simulink model "Emergency_Power_System"  (R2021b)
settings: Solver=FixedStepDiscrete  StartTime=0.0  StopTime=0.05  RelTol=1e-3
undefined symbols (not defined in the file): Ion, Lithium
libraries: spsSeriesRLCBranchLib x4, spsBatteryLib x1, spsBuckConverterLib x1, spsCurrentMeasurementLib x1, spsGroundLib x1, spsPWMGeneratorDCDCLib x1, spsVoltageMeasurementLib x1, spspowerguiLib x1
settings Model: Creator=KennyBoum-biha  LastModifiedBy=KennyBoum-biha

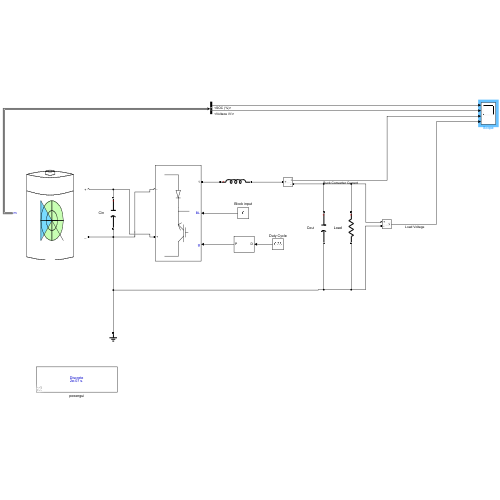
[thumbnail: Simulink's stored preview of the top-level diagram]
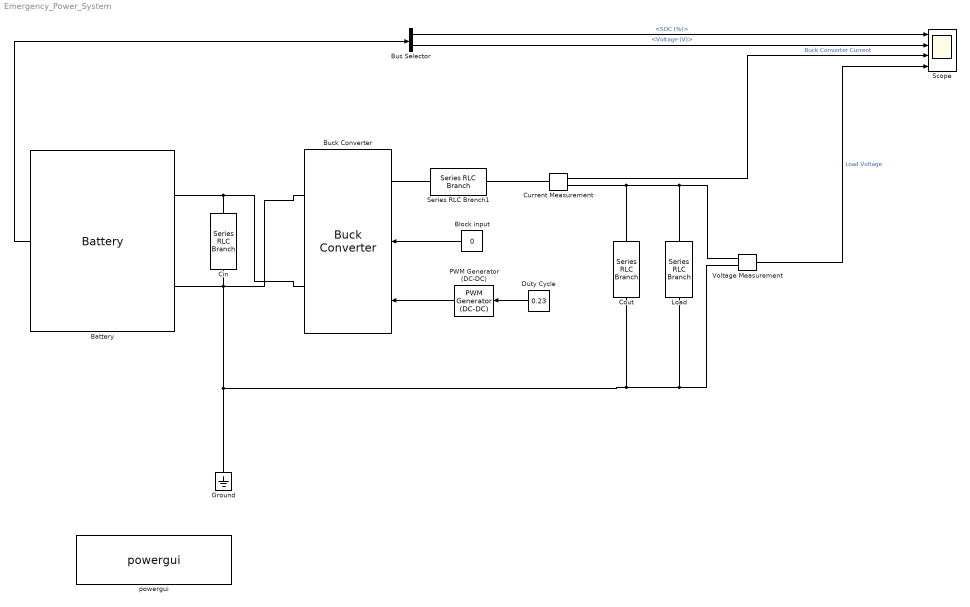
== system Emergency_Power_System ==
  Battery : spsBatteryLib/Battery  BatType=Lithium-Ion  ShowTempParam=off  ThermalPreset=no  ShowAgeParam=off  NomV=48  NomQ=10  SOC=80  Batt_Tr=0  PresetModel=on  MaxQ=10  MinV=36  FullV=55.8714  Dis_rate=4.3478  R=0.048  Normal_OP=9.0435  expZone="[51.8585     0.491304]"  current=[6.5 13 32.5]  Units=Time  Tci=20  NomT=20  T2=-30  MaxQ2=4.8  FullV2=7.1  Normal_OP2=5.655  expZone2="[6.58           1]"  Rca=0.6  ti=2000  Dp=0  Neq0=0  Tsim=1e6  Ta1=25  Qeol=5.4*0.9  Reol=0.013333*1.2  Char_age=[2.3478, 3]  Dis_age=[2.3478, 10]  N1=1500  N2=10500  N3=1000  N4=1400  Ta2=45  N5=950
  Block input : Constant  Value=0
  Buck Converter : spsBuckConverterLib/Buck Converter  ModelType=Switching devices  Ron=1e-3  Rs=1e6  Cs=inf  Vforward=[0,0]  Ron_Diode=1e-3  Rs_Diode=1e6  Cs_Diode=inf  Vf_Diode=1e-3  Rs_CurrentSource=inf
      settings: SourceProductBaseCode=PS
  Bus Selector : BusSelector  OutputSignals=SOC (%),Voltage (V)
  Cin : spsSeriesRLCBranchLib/Series RLC Branch  LConnTagsString=__new0  RConnTagsString=__new0  BranchType=C  Resistance=1  Inductance=1e-3  SetiL0=off  InitialCurrent=0  Capacitance=100e-6  Setx0=off  InitialVoltage=0  Measurements=None
  Cout : spsSeriesRLCBranchLib/Series RLC Branch  LConnTagsString=__new0  RConnTagsString=__new0  BranchType=C  Resistance=1  Inductance=1e-3  SetiL0=off  InitialCurrent=0  Capacitance=220e-6  Setx0=off  InitialVoltage=0  Measurements=None
  Current Measurement : spsCurrentMeasurementLib/Current Measurement  PhasorSimulation=off  OutputType=Complex  PSBequivalent=0
  Duty Cycle : Constant  Value=0.23
  Ground : spsGroundLib/Ground  LConnTagsString=a
  Load : spsSeriesRLCBranchLib/Series RLC Branch  LConnTagsString=__new0  RConnTagsString=__new0  BranchType=R  Resistance=1.44  Inductance=1e-3  SetiL0=off  InitialCurrent=0  Capacitance=1e-6  Setx0=off  InitialVoltage=0  Measurements=None
  PWM Generator (DC-DC) : spsPWMGeneratorDCDCLib/PWM Generator (DC-DC)  Fsw=50e3  Ts=2e-7
  Scope : Scope  NumInputPorts=4
  Series RLC Branch1 : spsSeriesRLCBranchLib/Series RLC Branch  LConnTagsString=__new0  RConnTagsString=__new0  BranchType=L  Resistance=1  Inductance=60e-6  SetiL0=off  InitialCurrent=0  Capacitance=1e-6  Setx0=off  InitialVoltage=0  Measurements=None
  Voltage Measurement : spsVoltageMeasurementLib/Voltage Measurement  PhasorSimulation=off  OutputType=Complex  PSBequivalent=0
  powergui : spspowerguiLib/powergui  Priority=1  SimulationMode=Discrete  SampleTime=2e-7  frequency=60  Iterations=50  frequencyindice=0  Pbase=100e6  ErrMax=1e-4  UnitsV=kV  UnitsW=MW  buscounter=0  FunctionMessages=off  echomessages=off  EnableUseOfTLC=off  CurrentSourceSwitches=off  DisableSnubberDevices=off  DisableRonSwitches=off  DisableVfSwitches=off  DisplayEquations=off  AutomaticDiscreteSolvers=off  SolverType=Tustin/Backward Euler (TBE)  Interpol=off  ExternalGateDelay=off  methode=off  Ts=100  x0status=blocks  SPID=on  SwTol=0  HookPort=off  NonlinearTolerance=1e-4  nMaxIteration=100  ContinueOnMaxIteration=off  RestoreLinks=warning  ResistiveCurrentMeasurement=off  Frange=[0:2:500]  Ylog=off  Xlog=on  ShowGrid=off  save=off  variable=ZData  structure=0  ZoomFFT=off  StartTime=0.0  cycles=1  DisplayStyle=1  fundamental=60  FreqAxis=off  MaxFrequency=1000  frequencyindicesteady=1  RmsSteady=1  display=off
  wires:
  PWM Generator (DC-DC)/1 -> Buck Converter/1
  Duty Cycle/1 -> PWM Generator (DC-DC)/1
  Block input/1 -> Buck Converter/2
  Current Measurement/1 -> Scope/3  "Buck Converter Current"
  Battery/1 -> Bus Selector/1
  Bus Selector/1 -> Scope/1  "<SOC (%)>"
  Bus Selector/2 -> Scope/2  "<Voltage (V)>"
  Voltage Measurement/1 -> Scope/4  "Load Voltage"
  connections:
  Current Measurement/LConn1 -- Series RLC Branch1/RConn1
  Ground/LConn1 -- Voltage Measurement/LConn2 -- Load/RConn1 -- Cout/RConn1 -- Cin/RConn1 -- Buck Converter/RConn2 -- Battery/LConn2
  Cin/LConn1 -- Buck Converter/RConn1 -- Battery/LConn1
  Series RLC Branch1/LConn1 -- Buck Converter/LConn1
  Current Measurement/RConn1 -- Voltage Measurement/LConn1 -- Load/LConn1 -- Cout/LConn1
